simulink library "copterFtc_lib"  (R2018b)
settings: Solver=VariableStepAuto  StartTime=0.0  StopTime=10.0  RelTol=1e-3
undefined symbols (not defined in the file): DiscIntNeverNeededParam, fm_loiter, simin
libraries: indi_lib x4, $bdroot x3, cntrlAttiRedIndi_lib x2, cntrlPosNdi_lib x1, axes_transformation_lib x1
settings Model: Creator=Ybeyer  LastModifiedBy=yannic
settings SFSimCC: SimUseLocalCustomCode=off
settings RTWCC: RTWUseLocalCustomCode=off
settings CodeAppCC: StateflowObjectComments=on

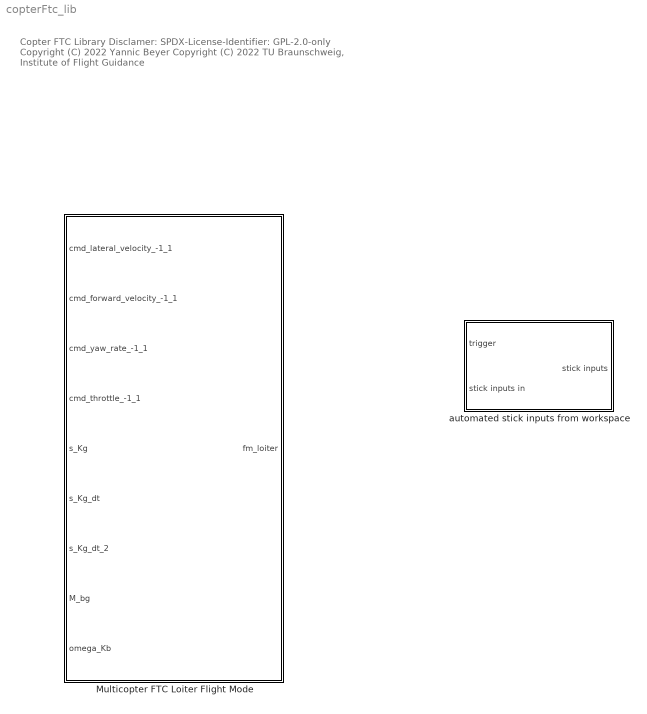
== system copterFtc_lib ==
  note: Copter FTC Library
      |
      | Disclamer:
      | SPDX-License-Identifier: GPL-2.0-only
      |
      | Copyright (C) 2022 Yannic Beyer
      | Copyright (C) 2022 TU Braunschweig, Institute of Flight Guidance
  Multicopter FTC Loiter Flight Mode : Subsystem  mask{fm=fm_loiter}
      mask prompts: fm "Multicopter INDI loiter flight  struct"
      mask DialogControl DescGroupVar Prompt: Multicopter INDI Loiter Flight Mode
      mask DialogControl DescTextVar Prompt: Loiter flight mode using the reduced attitude controller with INDI.
      mask DialogControl Control2 Prompt: To intialize the parameters struct see multicopterFlightModeLoiter.
  automated stick inputs from workspace : Subsystem  mask{simin=simin}
      mask prompts: simin "simin struct"
      mask DialogControl DescGroupVar Prompt: Automated stick inputs from workspace
      mask DialogControl DescTextVar Prompt: The stick inputs must be defined as a struct for the standard block "from workspace".

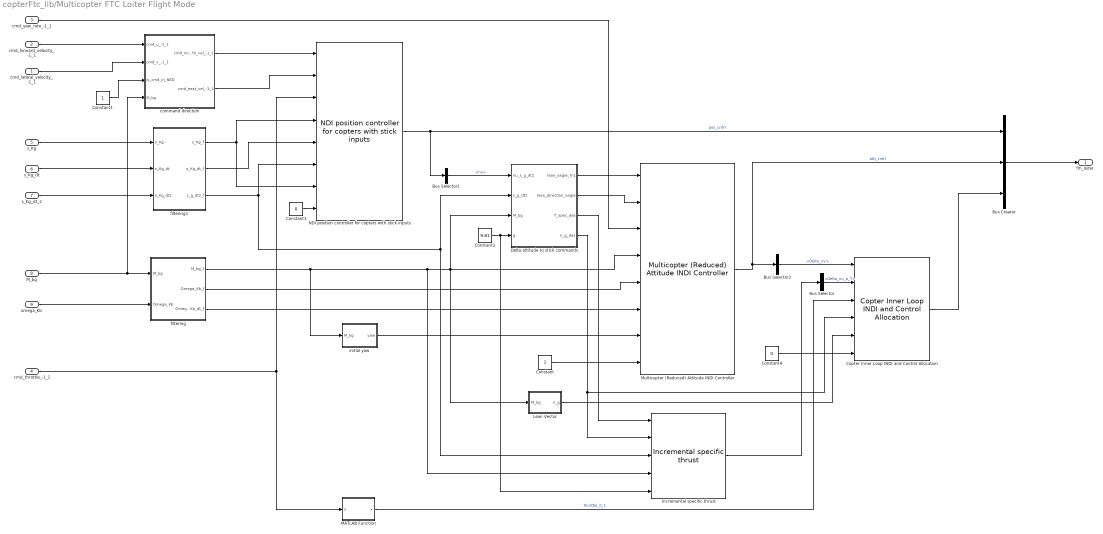
== system copterFtc_lib/Multicopter FTC Loiter Flight Mode ==
  cmd_lateral_velocity_-1_1 : Inport  SampleTime=double(fm.ts)
  cmd_forward_velocity_-1_1 : Inport  Port=2  SampleTime=double(fm.ts)
  cmd_yaw_rate_-1_1 : Inport  Port=3  SampleTime=double(fm.ts)
  cmd_throttle_-1_1 : Inport  Port=4  SampleTime=double(fm.ts)
  s_Kg : Inport  Port=5  SampleTime=double(fm.ts)
  s_Kg_dt : Inport  Port=6  SampleTime=double(fm.ts)
  s_Kg_dt_2 : Inport  Port=7  SampleTime=double(fm.ts)
  M_bg : Inport  Port=8  SampleTime=double(fm.ts)
  omega_Kb : Inport  Port=9  SampleTime=double(fm.ts)
  Bus Creator : BusCreator  Inputs=3
  Bus Selector : BusSelector  OutputSignals=Delta_nu_a_T
  Bus Selector1 : BusSelector  OutputSignals=pseudo_control.nu
  Bus Selector2 : BusSelector  OutputSignals=pseudo_control.Delta_ny
  Constant : Constant
  Constant1 : Constant
  Constant2 : Constant  Value=9.81
  Constant3 : Constant  Value=0
  Constant4 : Constant  Value=0
  Copter Inner Loop INDI and Control Allocation : indi_lib/Copter Inner Loop INDI and Control Allocation  cep=fm.cep  ceb=fm.ceb  ca=fm.ca  mtc=fm.mtc  sflt=fm.sflt  ts=fm.ts  is_ce_extern=off
      settings: SourceProductName=LADAC
  Delta attitude to stick commands : Subsystem
  Incremental specific thrust : indi_lib/Incremental specific thrust  leanfreq=fm.atc.rm.leanfreq  leandamp=fm.atc.rm.leandamp  is_enable_checked=off  states_when_enabling=held
      settings: SourceProductName=LADAC
  Lean Vector : MATLAB Function  TreatAsAtomicUnit=on
  MATLAB Function : MATLAB Function  TreatAsAtomicUnit=on
  Multicopter (Reduced) Attitude INDI Controller : cntrlAttiRedIndi_lib/Multicopter (Reduced) Attitude INDI Controller  atc=fm.atc  T=fm.mtc + 2./fm.sflt.omega
      settings: SourceProductName=LADAC
  NDI position controller for copters with stick inputs : cntrlPosNdi_lib/NDI position controller for copters with stick inputs  psc=fm.psc  T_inner_loop=2./fm.atc.rm.leanfreq + fm.mtc + 2./fm.sflt.omega  is_enable_checked=off  states_when_enabling=held
      settings: SourceProductName=LADAC
  command direction : Subsystem
  filtering : Subsystem
  filtering1 : Subsystem
  initial yaw : Subsystem
  fm_loiter : Outport  SampleTime=double(fm.ts)
  wires:
  Lean Vector/1(n_g) -> Copter Inner Loop INDI and Control Allocation/5
  cmd_forward_velocity_-1_1/1 -> command direction/1(cmd_u_-1_1)
  filtering1/2(s_Kg_dt_f) -> NDI position controller for copters with stick inputs/5
  filtering1/3(s_g_dt2_f) -> Incremental specific thrust/3, Delta attitude to stick commands/2(s_g_dt2), NDI position controller for copters with stick inputs/6
  cmd_yaw_rate_-1_1/1 -> Multicopter (Reduced) Attitude INDI Controller/3
  Constant/1 -> Multicopter (Reduced) Attitude INDI Controller/8
  filtering1/1(s_Kg_f) -> NDI position controller for copters with stick inputs/7, NDI position controller for copters with stick inputs/4
  filtering/2(Omega_Kb_f) -> Multicopter (Reduced) Attitude INDI Controller/5
  NDI position controller for copters with stick inputs/1 -> Bus Selector1/1, Bus Creator/1  "pos_cntrl"
  filtering/1(M_bg_f) -> Incremental specific thrust/4, Multicopter (Reduced) Attitude INDI Controller/4, Delta attitude to stick commands/3(M_bg), Lean Vector/1(M_bg), initial yaw/1(M_bg)
  cmd_lateral_velocity_-1_1/1 -> command direction/2(cmd_v_-1_1)
  Constant1/1 -> command direction/3(is_cmd_in_NED)
  Bus Selector1/1 -> Delta attitude to stick commands/1(nu_s_g_dt2)  "<nu>"
  Bus Creator/1 -> fm_loiter/1
  command direction/1(cmd_north_vel_-1_1) -> NDI position controller for copters with stick inputs/1
  command direction/2(cmd_east_vel_-1_1) -> NDI position controller for copters with stick inputs/2
  Multicopter (Reduced) Attitude INDI Controller/1 -> Bus Creator/2, Bus Selector2/1  "atti_cntrl"
  filtering/3(Omega_Kb_dt_f) -> Multicopter (Reduced) Attitude INDI Controller/6
  Delta attitude to stick commands/2(lean_direction_angle) -> Multicopter (Reduced) Attitude INDI Controller/2
  Delta attitude to stick commands/1(lean_angle_0-1) -> Multicopter (Reduced) Attitude INDI Controller/1
  MATLAB Function/1(y) -> Copter Inner Loop INDI and Control Allocation/3  "throttle_0_1"
  cmd_throttle_-1_1/1 -> NDI position controller for copters with stick inputs/3, MATLAB Function/1(u)
  Bus Selector2/1 -> Copter Inner Loop INDI and Control Allocation/1  "<Delta_ny>"
  Incremental specific thrust/1 -> Bus Selector/1
  Constant2/1 -> Incremental specific thrust/5, Delta attitude to stick commands/4(g)
  initial yaw/1(yaw) -> Multicopter (Reduced) Attitude INDI Controller/7
  Delta attitude to stick commands/3(T_spec_des) -> Incremental specific thrust/1
  Constant3/1 -> NDI position controller for copters with stick inputs/8
  s_Kg/1 -> filtering1/1(s_Kg)
  s_Kg_dt/1 -> filtering1/2(s_Kg_dt)
  s_Kg_dt_2/1 -> filtering1/3(s_Kg_dt2)
  M_bg/1 -> command direction/4(M_bg), filtering/1(M_bg)
  omega_Kb/1 -> filtering/2(Omega_Kb)
  Copter Inner Loop INDI and Control Allocation/1 -> Bus Creator/3
  Delta attitude to stick commands/4(n_g_des) -> Copter Inner Loop INDI and Control Allocation/4, Incremental specific thrust/2
  Constant4/1 -> Copter Inner Loop INDI and Control Allocation/6
  Bus Selector/1 -> Copter Inner Loop INDI and Control Allocation/2  "<Delta_nu_a_T>"

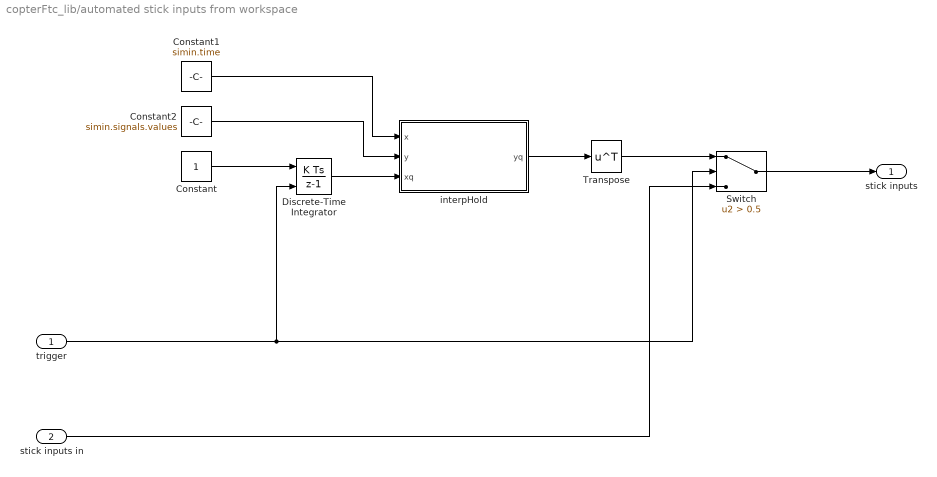
== system copterFtc_lib/automated stick inputs from workspace ==
  trigger : Inport
  stick inputs in : Inport  Port=2
  Constant : Constant
  Constant1 : Constant  Value=simin.time
  Constant2 : Constant  Value=simin.signals.values
  Discrete-Time Integrator : DiscreteIntegrator  ExternalReset=rising  SampleTime=-1  ICPrevOutput=DiscIntNeverNeededParam  ICPrevScaledInput=DiscIntNeverNeededParam
  Switch : Switch  Criteria=u2 > Threshold  Threshold=0.5
  Transpose : Math  Operator=transpose  SaturateOnIntegerOverflow=on
  interpHold : MATLAB Function  TreatAsAtomicUnit=on
  stick inputs : Outport
  wires:
  Constant1/1 -> interpHold/1(x)
  Discrete-Time Integrator/1 -> interpHold/3(xq)
  interpHold/1(yq) -> Transpose/1
  Constant2/1 -> interpHold/2(y)
  Constant/1 -> Discrete-Time Integrator/1
  Switch/1 -> stick inputs/1
  stick inputs in/1 -> Switch/3
  Transpose/1 -> Switch/1
  trigger/1 -> Switch/2, Discrete-Time Integrator/2

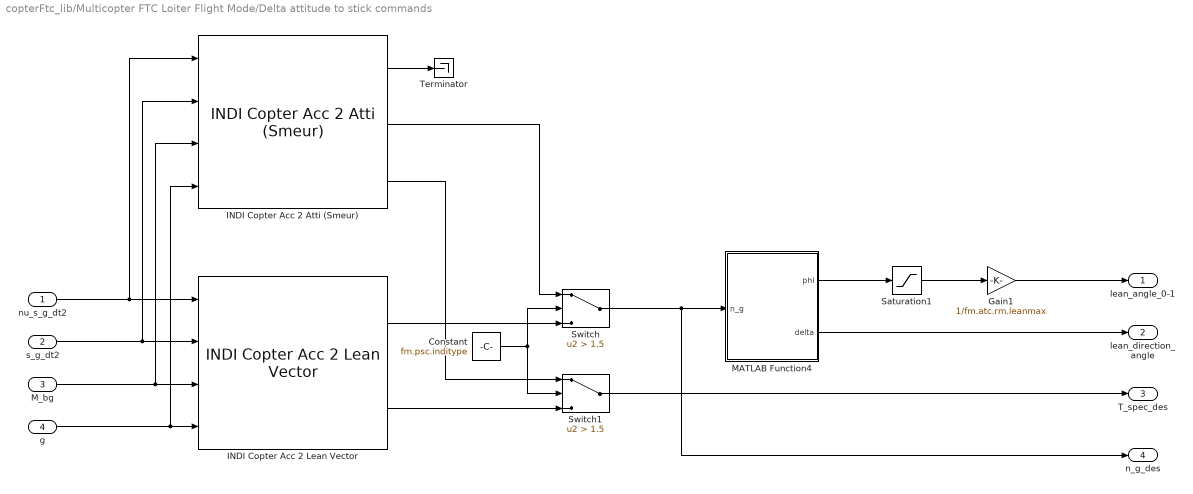
== system copterFtc_lib/Multicopter FTC Loiter Flight Mode/Delta attitude to stick commands ==
  nu_s_g_dt2 : Inport
  s_g_dt2 : Inport  Port=2
  M_bg : Inport  Port=3
  g : Inport  Port=4
  Constant : Constant  Value=fm.psc.inditype
  Gain1 : Gain  Gain=1/fm.atc.rm.leanmax
  INDI Copter Acc 2 Atti (Smeur) : indi_lib/INDI Copter Acc 2 Atti (Smeur)  SystemSampleTime=-1
      settings: SourceProductName=LADAC
  INDI Copter Acc 2 Lean Vector : indi_lib/INDI Copter Acc 2 Lean Vector  SystemSampleTime=-1
      settings: SourceProductName=LADAC
  MATLAB Function4 : MATLAB Function  TreatAsAtomicUnit=on
  Saturation1 : Saturate  UpperLimit=fm.atc.rm.leanmax  LowerLimit=0
  Switch : Switch  Criteria=u2 > Threshold  Threshold=1.5
  Switch1 : Switch  Criteria=u2 > Threshold  Threshold=1.5
  Terminator : Terminator
  lean_angle_0-1 : Outport
  lean_direction_angle : Outport  Port=2
  T_spec_des : Outport  Port=3
  n_g_des : Outport  Port=4
  wires:
  Constant/1 -> Switch/2, Switch1/2
  INDI Copter Acc 2 Atti (Smeur)/3 -> Switch1/1
  INDI Copter Acc 2 Lean Vector/2 -> Switch1/3
  INDI Copter Acc 2 Lean Vector/1 -> Switch/3
  INDI Copter Acc 2 Atti (Smeur)/2 -> Switch/1
  INDI Copter Acc 2 Atti (Smeur)/1 -> Terminator/1
  Switch1/1 -> T_spec_des/1
  M_bg/1 -> INDI Copter Acc 2 Lean Vector/3, INDI Copter Acc 2 Atti (Smeur)/3
  s_g_dt2/1 -> INDI Copter Acc 2 Atti (Smeur)/2, INDI Copter Acc 2 Lean Vector/2
  g/1 -> INDI Copter Acc 2 Lean Vector/4, INDI Copter Acc 2 Atti (Smeur)/4
  MATLAB Function4/1(phi) -> Saturation1/1
  Saturation1/1 -> Gain1/1
  nu_s_g_dt2/1 -> INDI Copter Acc 2 Atti (Smeur)/1, INDI Copter Acc 2 Lean Vector/1
  Gain1/1 -> lean_angle_0-1/1
  MATLAB Function4/2(delta) -> lean_direction_angle/1
  Switch/1 -> n_g_des/1, MATLAB Function4/1(n_g)

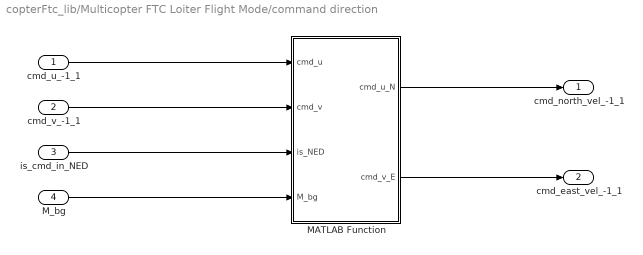
== system copterFtc_lib/Multicopter FTC Loiter Flight Mode/command direction ==
  cmd_u_-1_1 : Inport
  cmd_v_-1_1 : Inport  Port=2
  is_cmd_in_NED : Inport  Port=3
  M_bg : Inport  Port=4
  MATLAB Function : MATLAB Function  TreatAsAtomicUnit=on
  cmd_north_vel_-1_1 : Outport
  cmd_east_vel_-1_1 : Outport  Port=2
  wires:
  cmd_u_-1_1/1 -> MATLAB Function/1(cmd_u)
  cmd_v_-1_1/1 -> MATLAB Function/2(cmd_v)
  is_cmd_in_NED/1 -> MATLAB Function/3(is_NED)
  MATLAB Function/1(cmd_u_N) -> cmd_north_vel_-1_1/1
  MATLAB Function/2(cmd_v_E) -> cmd_east_vel_-1_1/1
  M_bg/1 -> MATLAB Function/4(M_bg)

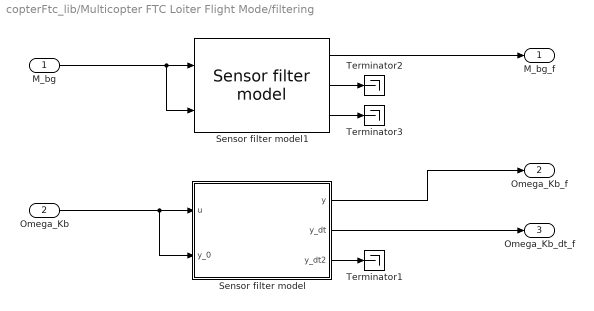
== system copterFtc_lib/Multicopter FTC Loiter Flight Mode/filtering ==
  M_bg : Inport
  Omega_Kb : Inport  Port=2
  Sensor filter model : Subsystem  mask{omega=fm.sflt.omega, d=fm.sflt.D, x_dt2_max=inf, x_dt2_min=-inf, x_dt_max=inf, x_dt_min=-inf, x_max=inf, x_min=-inf, x_init=0, x_dt_init=0}
      mask prompts: omega "Natural frequency"; d "Damping ratio"; x_dt2_max "Maximum acceleration"; x_dt2_min "Minimum acceleration"; x_dt_max "Maximum rate"; x_dt_min "Minimum rate"; x_max "Maximum position"; x_min "Minimum position"; x_init "Initial position"; x_dt_init "Initial rate"
  Sensor filter model1 : $bdroot/Multicopter FTC Loiter Flight Mode/filtering/Sensor filter model  omega=fm.sflt.omega  d=fm.sflt.D  x_dt2_max=inf  x_dt2_min=-inf  x_dt_max=inf  x_dt_min=-inf  x_max=inf  x_min=-inf  x_init=0  x_dt_init=0
  Terminator1 : Terminator
  Terminator2 : Terminator
  Terminator3 : Terminator
  M_bg_f : Outport
  Omega_Kb_f : Outport  Port=2
  Omega_Kb_dt_f : Outport  Port=3
  wires:
  Sensor filter model/3(y_dt2) -> Terminator1/1
  Sensor filter model/2(y_dt) -> Omega_Kb_dt_f/1
  Omega_Kb/1 -> Sensor filter model/2(y_0), Sensor filter model/1(u)
  Sensor filter model/1(y) -> Omega_Kb_f/1
  M_bg/1 -> Sensor filter model1/1, Sensor filter model1/2
  Sensor filter model1/1 -> M_bg_f/1
  Sensor filter model1/2 -> Terminator2/1
  Sensor filter model1/3 -> Terminator3/1

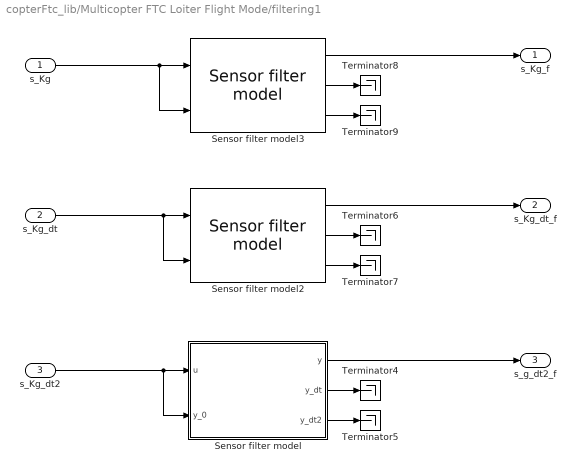
== system copterFtc_lib/Multicopter FTC Loiter Flight Mode/filtering1 ==
  s_Kg : Inport
  s_Kg_dt : Inport  Port=2
  s_Kg_dt2 : Inport  Port=3
  Sensor filter model : Subsystem  mask{omega=fm.sflt.omega, d=fm.sflt.D, x_dt2_max=inf, x_dt2_min=-inf, x_dt_max=inf, x_dt_min=-inf, x_max=inf, x_min=-inf, x_init=0, x_dt_init=0}
      mask prompts: omega "Natural frequency"; d "Damping ratio"; x_dt2_max "Maximum acceleration"; x_dt2_min "Minimum acceleration"; x_dt_max "Maximum rate"; x_dt_min "Minimum rate"; x_max "Maximum position"; x_min "Minimum position"; x_init "Initial position"; x_dt_init "Initial rate"
  Sensor filter model2 : $bdroot/Multicopter FTC Loiter Flight Mode/filtering1/Sensor filter model  omega=fm.sflt.omega  d=fm.sflt.D  x_dt2_max=inf  x_dt2_min=-inf  x_dt_max=inf  x_dt_min=-inf  x_max=inf  x_min=-inf  x_init=0  x_dt_init=0
  Sensor filter model3 : $bdroot/Multicopter FTC Loiter Flight Mode/filtering1/Sensor filter model  omega=fm.sflt.omega  d=fm.sflt.D  x_dt2_max=inf  x_dt2_min=-inf  x_dt_max=inf  x_dt_min=-inf  x_max=inf  x_min=-inf  x_init=0  x_dt_init=0
  Terminator{4..9} (6 alike) : Terminator
  s_Kg_f : Outport
  s_Kg_dt_f : Outport  Port=2
  s_g_dt2_f : Outport  Port=3
  wires:
  s_Kg/1 -> Sensor filter model3/1, Sensor filter model3/2
  Sensor filter model3/3 -> Terminator9/1
  Sensor filter model3/2 -> Terminator8/1
  Sensor filter model3/1 -> s_Kg_f/1
  Sensor filter model2/3 -> Terminator7/1
  Sensor filter model2/2 -> Terminator6/1
  s_Kg_dt/1 -> Sensor filter model2/2, Sensor filter model2/1
  Sensor filter model2/1 -> s_Kg_dt_f/1
  Sensor filter model/3(y_dt2) -> Terminator5/1
  Sensor filter model/2(y_dt) -> Terminator4/1
  s_Kg_dt2/1 -> Sensor filter model/1(u), Sensor filter model/2(y_0)
  Sensor filter model/1(y) -> s_g_dt2_f/1

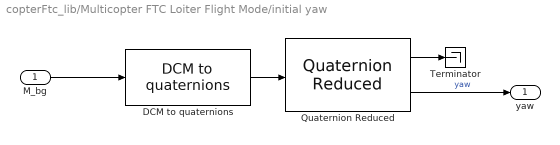
== system copterFtc_lib/Multicopter FTC Loiter Flight Mode/initial yaw ==
  M_bg : Inport
  DCM to quaternions : axes_transformation_lib/DCM to quaternions  SystemSampleTime=-1
      settings: SourceProductName=LADAC
  Quaternion Reduced : cntrlAttiRedIndi_lib/Multicopter (Reduced) Attitude INDI Controller/measure/Quaternion Reduced  SystemSampleTime=-1
      settings: SourceProductName=LADAC
  Terminator : Terminator
  yaw : Outport
  wires:
  DCM to quaternions/1 -> Quaternion Reduced/1
  M_bg/1 -> DCM to quaternions/1
  Quaternion Reduced/2 -> yaw/1  "yaw"
  Quaternion Reduced/1 -> Terminator/1

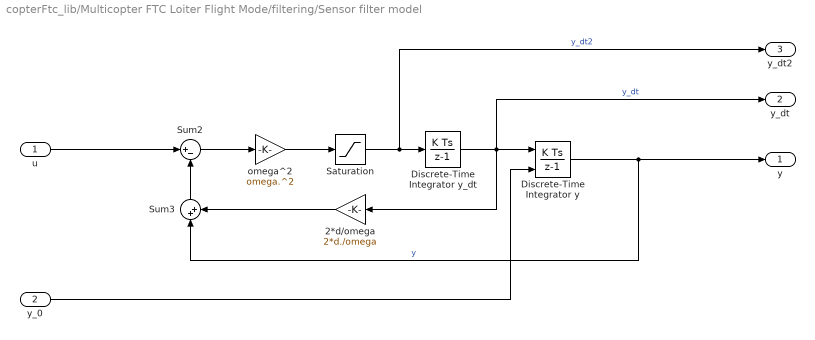
== system copterFtc_lib/Multicopter FTC Loiter Flight Mode/filtering/Sensor filter model ==
  u : Inport
  y_0 : Inport  Port=2
  2*d/omega : Gain  Gain=2*d./omega
  Discrete-Time Integrator y : DiscreteIntegrator  InitialConditionSource=external  InitialCondition=x_init  SampleTime=-1  LimitOutput=on  UpperSaturationLimit=x_max  LowerSaturationLimit=x_min  ICPrevOutput=DiscIntNeverNeededParam  ICPrevScaledInput=DiscIntNeverNeededParam
  Discrete-Time Integrator y_dt : DiscreteIntegrator  InitialCondition=x_dt_init  SampleTime=-1  LimitOutput=on  UpperSaturationLimit=x_dt_max  LowerSaturationLimit=x_dt_min  ICPrevOutput=DiscIntNeverNeededParam  ICPrevScaledInput=DiscIntNeverNeededParam
  Saturation : Saturate  UpperLimit=x_dt2_max  LowerLimit=x_dt2_min
  Sum2 : Sum  Inputs=|+-
  Sum3 : Sum  Inputs=|++
  omega^2 : Gain  Gain=omega.^2
  y : Outport
  y_dt : Outport  Port=2
  y_dt2 : Outport  Port=3
  wires:
  Saturation/1 -> y_dt2/1, Discrete-Time Integrator y_dt/1  "y_dt2"
  omega^2/1 -> Saturation/1
  Sum3/1 -> Sum2/2
  u/1 -> Sum2/1
  2*d/omega/1 -> Sum3/2
  Sum2/1 -> omega^2/1
  Discrete-Time Integrator y/1 -> y/1, Sum3/1  "y"
  Discrete-Time Integrator y_dt/1 -> 2*d/omega/1, y_dt/1, Discrete-Time Integrator y/1  "y_dt"
  y_0/1 -> Discrete-Time Integrator y/2

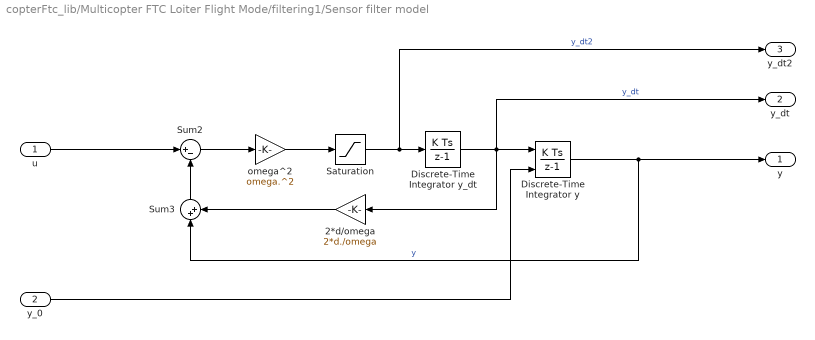
== system copterFtc_lib/Multicopter FTC Loiter Flight Mode/filtering1/Sensor filter model ==
  u : Inport
  y_0 : Inport  Port=2
  2*d/omega : Gain  Gain=2*d./omega
  Discrete-Time Integrator y : DiscreteIntegrator  InitialConditionSource=external  InitialCondition=x_init  SampleTime=-1  LimitOutput=on  UpperSaturationLimit=x_max  LowerSaturationLimit=x_min  ICPrevOutput=DiscIntNeverNeededParam  ICPrevScaledInput=DiscIntNeverNeededParam
  Discrete-Time Integrator y_dt : DiscreteIntegrator  InitialCondition=x_dt_init  SampleTime=-1  LimitOutput=on  UpperSaturationLimit=x_dt_max  LowerSaturationLimit=x_dt_min  ICPrevOutput=DiscIntNeverNeededParam  ICPrevScaledInput=DiscIntNeverNeededParam
  Saturation : Saturate  UpperLimit=x_dt2_max  LowerLimit=x_dt2_min
  Sum2 : Sum  Inputs=|+-
  Sum3 : Sum  Inputs=|++
  omega^2 : Gain  Gain=omega.^2
  y : Outport
  y_dt : Outport  Port=2
  y_dt2 : Outport  Port=3
  wires:
  y_0/1 -> Discrete-Time Integrator y/2
  Discrete-Time Integrator y_dt/1 -> Discrete-Time Integrator y/1, y_dt/1, 2*d/omega/1  "y_dt"
  Discrete-Time Integrator y/1 -> Sum3/1, y/1  "y"
  Sum2/1 -> omega^2/1
  2*d/omega/1 -> Sum3/2
  u/1 -> Sum2/1
  Sum3/1 -> Sum2/2
  omega^2/1 -> Saturation/1
  Saturation/1 -> Discrete-Time Integrator y_dt/1, y_dt2/1  "y_dt2"

== matlab function copterFtc_lib/Multicopter FTC Loiter Flight Mode/command direction/MATLAB Function ==
  data: cmd_u input; cmd_u_N output; cmd_v input; is_NED input; cmd_v_E output; M_bg input
function [cmd_u_N,cmd_v_E] = fcn( cmd_u, cmd_v, is_NED, M_bg )

if is_NED
    cmd_u_N = cmd_u;
    cmd_v_E = cmd_v;
else
    EulerAngle = dcm2Euler(M_bg);
    yaw = EulerAngle(3);
    M_NED_FRD = euler2Dcm([0;0;yaw])';
    cmd_V_NED = M_NED_FRD * [ cmd_u; cmd_v; 0 ];
    cmd_u_N = cmd_V_NED(1);
    cmd_v_E = cmd_V_NED(2);
end

end

== matlab function copterFtc_lib/Multicopter FTC Loiter Flight Mode/Delta attitude to stick commands/MATLAB Function4 ==
  data: n_g input; phi output; delta output
function [phi,delta] = leanVector2LeanAngles(n_g)
[phi,delta] = leanVector2LeanAngles(n_g);
end

== matlab function copterFtc_lib/Multicopter FTC Loiter Flight Mode/MATLAB Function ==
  data: u input; y output
function y = fcn(u)
y = 0.5*u+0.5;

== matlab function copterFtc_lib/automated stick inputs from workspace/interpHold ==
  data: x input; yq output; y input; xq input
function yq = interpHold( x, y, xq )
yq = interpHold( x, y, xq );
end

== matlab function copterFtc_lib/Multicopter FTC Loiter Flight Mode/Lean Vector ==
  data: M_bg input; n_g output
function n_g = fcn(M_bg)
n_g = dcm2LeanVector(M_bg);
end
